simulink model "solar_tracker"  (R2024b)
settings: Solver=FixedStepDiscrete  StartTime=0.0  StopTime=10.0  FixedStep=0.2  RelTol=1e-3
undefined symbols (not defined in the file): u_max, u_min
settings Model: Creator=Ali Saleh Al-Taher  LastModifiedBy=Ali Saleh Al-Taher

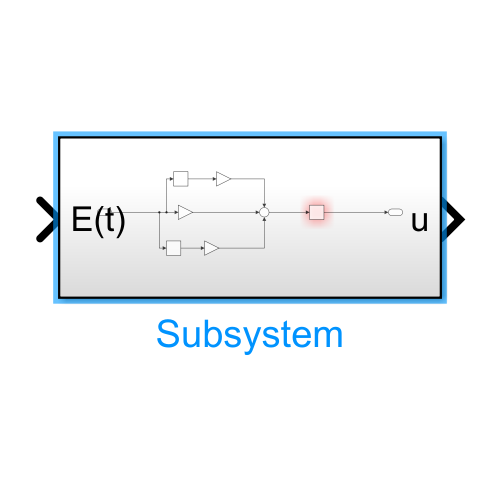
[thumbnail: Simulink's stored preview of the top-level diagram]
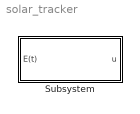
== system solar_tracker ==
  Subsystem : Subsystem

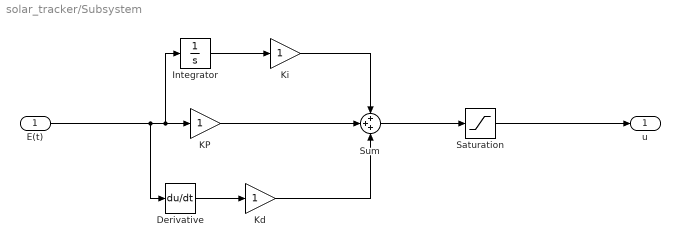
== system solar_tracker/Subsystem ==
  E(t) : Inport
  Derivative : Derivative
  Integrator : Integrator
  KP : Gain
  Kd : Gain
  Ki : Gain
  Saturation : Saturate  UpperLimit=u_max  LowerLimit=u_min
  Sum : Sum  Inputs=+++
  u : Outport
  wires:
  Integrator/1 -> Ki/1
  E(t)/1 -> Derivative/1, Integrator/1, KP/1
  Derivative/1 -> Kd/1
  KP/1 -> Sum/2
  Kd/1 -> Sum/3
  Ki/1 -> Sum/1
  Saturation/1 -> u/1
  Sum/1 -> Saturation/1
